simulink model "TestDistancia"  (R2022b)
settings: Solver=FixedStepAuto  StartTime=0.0  StopTime=inf  RelTol=1e-3  EnableMultiTasking=on
settings Model: ExtModeTrigDuration=2  Creator=miriamfreiriasanjuan  LastModifiedBy=miriamfreiriasanjuan
settings OptimizationCC: EnhancedBackFolding=on  PassReuseOutputArgsAs=Individual arguments  ZeroExternalMemoryAtStartup=off  ZeroInternalMemoryAtStartup=off  MaxStackSize=64  OptimizeBlockOrder=speed  DifferentSizesBufferReuse=on  OptimizationCustomize=off  EfficientTunableParamExpr=on
settings DebuggingCC: ParameterOverflowMsg=none  ParameterTunabilityLossMsg=error
settings HardwareCC: ProdBitPerInt=16  ProdBitPerPointer=16  ProdBitPerSizeT=16  ProdBitPerPtrDiffT=16  ProdLargestAtomicFloat=None  ProdWordSize=8  ProdHWDeviceType=Atmel->AVR
settings SFSimCC: MATLABDynamicMemAlloc=off
settings RTWCC: Description=Embedded Coder  SystemTargetFile=ert.tlc  HardwareBoard=Arduino Mega 2560  TLCOptions=-aInlineSetEventsForThisBaseRateFcn=TLC_FALSE -aSuppressMultiTaskScheduler=TLC_FALSE -aRateBasedStepFcn=1  TemplateMakefile=ert_default_tmf  Toolchain=Arduino AVR  BuildConfiguration=Faster Runs
settings CodeAppCC: ForceParamTrailComments=on  IgnoreCustomStorageClasses=off  OperatorAnnotations=on  SimulinkDataObjDesc=on  SFDataObjDesc=on  InsertBlockDesc=on
settings ERTTargetCC: SupportContinuousTime=on  SupportVariableSizeSignals=on  ExtModeTransport=3  ExtModeStaticAlloc=on  ExtModeAutomaticAllocSize=off  ExtModeStaticAllocSize=2048  ExtModeMexFile=ext_xcp  ExtModeIntrfLevel=Level2 - Open

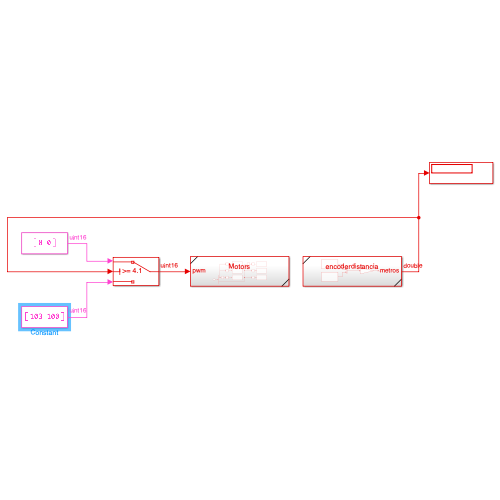
[thumbnail: Simulink's stored preview of the top-level diagram]
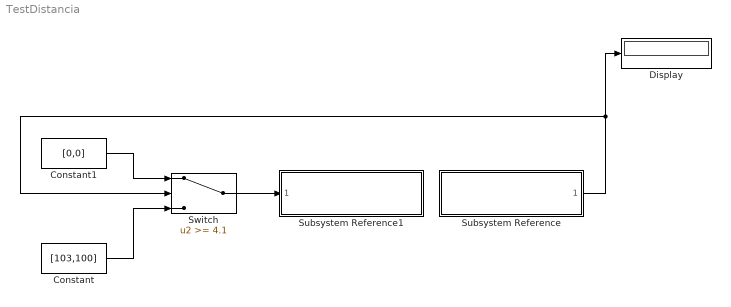
== system TestDistancia ==
  Constant : Constant  Value=[103,100]  OutDataTypeStr=uint16
  Constant1 : Constant  Value=[0,0]  OutMin=0  OutMax=0  OutDataTypeStr=uint16
  Display : Display
  Subsystem Reference : Subsystem  ReferencedSubsystem=encoderdistancia
  Subsystem Reference1 : Subsystem  ReferencedSubsystem=Motors
  Switch : Switch  Threshold=4.1  SaturateOnIntegerOverflow=off  InputSameDT=off
  wires:
  Subsystem Reference/1 -> Display/1, Switch/2
  Constant1/1 -> Switch/1
  Constant/1 -> Switch/3
  Switch/1 -> Subsystem Reference1/1
